simulink library "sm_wheel_loader_lib"  (R2025a)
settings: Solver=VariableStepAuto  StartTime=0.0  StopTime=10.0  RelTol=1e-3
undefined symbols (not defined in the file): AToTOrificeVector, BiPOrificeVector, boomHEArea, boomREArea, BToTOrificeVector, fluids, GRake, GToothL, GToothR, HMPST, HydFcnParams, logLoad, Position, PToAOrificeVector, PToBOrificeVector, RakeL, RakeR, testInput, Wheel_Loader, X, Y, Z
libraries: sm_lib x694, fl_lib x183, nesl_utility x74, SimscapeFluids_lib x62, sdl_lib x25, cvt_components_lib x25, simulink_extras x5, $bdroot x4, wheel_loader_contact_lib x4, ee_lib x2, SignalEditorBlockLib x1, batteryecm_lib x1
(part 9 of 26)

== system sm_wheel_loader_lib/Wheel Loader Vehicle/Load/Log ==
  Load : Inport
  Base : Subsystem  mask{TranslationCartesianOffset=base_location, RotationAngle=base_orientation}
      mask prompts: TranslationCartesianOffset "Location Base [x y z] (m)"; RotationAngle "Orientation Base (deg)"
      mask TypeOptions TranslationCartesianOffset:
      | Transform
      | Location Base/TranslationCartesianOffset
      mask TypeOptions RotationAngle:
      | Transform
      | Orient Base/RotationAngle
      mask Display: image('sm_wheel_loader_logbase_IMAGE.png')
  Bin : Subsystem  mask{TranslationCartesianOffset=bin_location, RotationAngle=bin_orientation}
      mask prompts: TranslationCartesianOffset "Bin Offset [x y z] (m)"; RotationAngle "Bin Orientation about z (deg)"
      mask TypeOptions TranslationCartesianOffset:
      | Transform
      | Location Base/TranslationCartesianOffset
      mask TypeOptions RotationAngle:
      | Transform
      | Orient Base/RotationAngle
      mask Display: image('sm_wheel_loader_logbin_IMAGE.png')
  Bushing Joint : sm_lib/Joints/Bushing Joint  JointMode=Normal  CompositeWrenchDir=FollowerOnBase  CompositeWrenchFrame=BaseFrame  SenseConstraintForce=off  SenseConstraintTorque=off  SenseTotalForce=off  SenseTotalTorque=off  PxPositionTargetSpecify=off  PxPositionTargetPriority=High  PxPositionTargetValue=0  PxPositionTargetValueUnits=m  PxVelocityTargetSpecify=off  PxVelocityTargetPriority=High  PxVelocityTargetValue=0  PxVelocityTargetValueUnits=m/s  PxEquilibriumPosition=0  PxEquilibriumPositionUnits=m  PxSpringStiffness=0  PxSpringStiffnessUnits=N/m  PxDampingCoefficient=0  PxDampingCoefficientUnits=N/(m/s)  PxLowerLimitSpecify=off  PxLowerLimitBound=-1  PxLowerLimitBoundUnits=m  PxLowerLimitStiffness=1e6  PxLowerLimitStiffnessUnits=N/m  PxLowerLimitDamping=1e3  PxLowerLimitDampingUnits=N/(m/s)  PxLowerLimitTransitionRegionWidth=1e-4  PxLowerLimitTransitionRegionWidthUnits=m  PxUpperLimitSpecify=off  PxUpperLimitBound=1  PxUpperLimitBoundUnits=m  PxUpperLimitStiffness=1e6  PxUpperLimitStiffnessUnits=N/m  PxUpperLimitDamping=1e3  PxUpperLimitDampingUnits=N/(m/s)  PxUpperLimitTransitionRegionWidth=1e-4  PxUpperLimitTransitionRegionWidthUnits=m  PxTorqueActuationMode=NoTorque  PxMotionActuationMode=ComputedMotion  PxSensePosition=off  PxSenseVelocity=off  PxSenseAcceleration=off  PxSenseTorqueForce=off  PxSenseLowerLimitTorqueForce=off  PxSenseUpperLimitTorqueForce=off  PyPositionTargetSpecify=off  PyPositionTargetPriority=High  PyPositionTargetValue=0  PyPositionTargetValueUnits=m  PyVelocityTargetSpecify=off  PyVelocityTargetPriority=High  PyVelocityTargetValue=0  PyVelocityTargetValueUnits=m/s  PyEquilibriumPosition=0  PyEquilibriumPositionUnits=m  PySpringStiffness=0  PySpringStiffnessUnits=N/m  PyDampingCoefficient=0  PyDampingCoefficientUnits=N/(m/s)  PyLowerLimitSpecify=off  PyLowerLimitBound=-1  PyLowerLimitBoundUnits=m  PyLowerLimitStiffness=1e6  PyLowerLimitStiffnessUnits=N/m  PyLowerLimitDamping=1e3  PyLowerLimitDampingUnits=N/(m/s)  PyLowerLimitTransitionRegionWidth=1e-4  PyLowerLimitTransitionRegionWidthUnits=m  PyUpperLimitSpecify=off  PyUpperLimitBound=1  PyUpperLimitBoundUnits=m  PyUpperLimitStiffness=1e6  PyUpperLimitStiffnessUnits=N/m  PyUpperLimitDamping=1e3  PyUpperLimitDampingUnits=N/(m/s)  PyUpperLimitTransitionRegionWidth=1e-4  PyUpperLimitTransitionRegionWidthUnits=m  PyTorqueActuationMode=NoTorque  PyMotionActuationMode=ComputedMotion  PySensePosition=off  PySenseVelocity=off  PySenseAcceleration=off  PySenseTorqueForce=off  PySenseLowerLimitTorqueForce=off  PySenseUpperLimitTorqueForce=off  PzPositionTargetSpecify=off  PzPositionTargetPriority=High  PzPositionTargetValue=0  PzPositionTargetValueUnits=m  PzVelocityTargetSpecify=off  PzVelocityTargetPriority=High  PzVelocityTargetValue=0  PzVelocityTargetValueUnits=m/s  PzEquilibriumPosition=0  PzEquilibriumPositionUnits=m  PzSpringStiffness=0  PzSpringStiffnessUnits=N/m  PzDampingCoefficient=0  PzDampingCoefficientUnits=N/(m/s)  PzLowerLimitSpecify=off  PzLowerLimitBound=-1  PzLowerLimitBoundUnits=m  PzLowerLimitStiffness=1e6  PzLowerLimitStiffnessUnits=N/m  PzLowerLimitDamping=1e3  PzLowerLimitDampingUnits=N/(m/s)  PzLowerLimitTransitionRegionWidth=1e-4  PzLowerLimitTransitionRegionWidthUnits=m  PzUpperLimitSpecify=off  PzUpperLimitBound=1  PzUpperLimitBoundUnits=m  PzUpperLimitStiffness=1e6  PzUpperLimitStiffnessUnits=N/m  PzUpperLimitDamping=1e3  PzUpperLimitDampingUnits=N/(m/s)  PzUpperLimitTransitionRegionWidth=1e-4  PzUpperLimitTransitionRegionWidthUnits=m  PzTorqueActuationMode=NoTorque  PzMotionActuationMode=ComputedMotion  PzSensePosition=off  PzSenseVelocity=off  PzSenseAcceleration=off  PzSenseTorqueForce=off  PzSenseLowerLimitTorqueForce=off  PzSenseUpperLimitTorqueForce=off  RxPositionTargetSpecify=off  RxPositionTargetPriority=High  RxPositionTargetValue=0  RxPositionTargetValueUnits=deg  RxVelocityTargetSpecify=off  RxVelocityTargetPriority=High  RxVelocityTargetValue=0  RxVelocityTargetValueUnits=deg/s  RxEquilibriumPosition=0  RxEquilibriumPositionUnits=deg  RxSpringStiffness=0  RxSpringStiffnessUnits=N*m/deg  RxDampingCoefficient=0  RxDampingCoefficientUnits=N*m/(deg/s)  RxLowerLimitSpecify=off  RxLowerLimitBound=-90  RxLowerLimitBoundUnits=deg  RxLowerLimitStiffness=1e4  RxLowerLimitStiffnessUnits=N*m/deg  RxLowerLimitDamping=10  RxLowerLimitDampingUnits=N*m/(deg/s)  RxLowerLimitTransitionRegionWidth=0.1  RxLowerLimitTransitionRegionWidthUnits=deg  RxUpperLimitSpecify=off  RxUpperLimitBound=90  RxUpperLimitBoundUnits=deg  RxUpperLimitStiffness=1e4  RxUpperLimitStiffnessUnits=N*m/deg  RxUpperLimitDamping=10  RxUpperLimitDampingUnits=N*m/(deg/s)  RxUpperLimitTransitionRegionWidth=0.1  RxUpperLimitTransitionRegionWidthUnits=deg  RxTorqueActuationMode=NoTorque  RxMotionActuationMode=ComputedMotion  RxSensePosition=off  RxSenseVelocity=off  RxSenseAcceleration=off  RxSenseTorqueForce=off  RxSenseLowerLimitTorqueForce=off  RxSenseUpperLimitTorqueForce=off  RyPositionTargetSpecify=off  RyPositionTargetPriority=High  RyPositionTargetValue=0  RyPositionTargetValueUnits=deg  RyVelocityTargetSpecify=off  RyVelocityTargetPriority=High  RyVelocityTargetValue=0  RyVelocityTargetValueUnits=deg/s  RyEquilibriumPosition=0  RyEquilibriumPositionUnits=deg  RySpringStiffness=0  RySpringStiffnessUnits=N*m/deg  RyDampingCoefficient=0  RyDampingCoefficientUnits=N*m/(deg/s)  RyLowerLimitSpecify=off  RyLowerLimitBound=-90  RyLowerLimitBoundUnits=deg  RyLowerLimitStiffness=1e4  RyLowerLimitStiffnessUnits=N*m/deg  RyLowerLimitDamping=10  RyLowerLimitDampingUnits=N*m/(deg/s)  RyLowerLimitTransitionRegionWidth=0.1  RyLowerLimitTransitionRegionWidthUnits=deg  RyUpperLimitSpecify=off  RyUpperLimitBound=90  RyUpperLimitBoundUnits=deg  RyUpperLimitStiffness=1e4  RyUpperLimitStiffnessUnits=N*m/deg  RyUpperLimitDamping=10  RyUpperLimitDampingUnits=N*m/(deg/s)  RyUpperLimitTransitionRegionWidth=0.1  RyUpperLimitTransitionRegionWidthUnits=deg  RyTorqueActuationMode=NoTorque  RyMotionActuationMode=ComputedMotion  RySensePosition=off  RySenseVelocity=off  RySenseAcceleration=off  RySenseTorqueForce=off  RySenseLowerLimitTorqueForce=off  RySenseUpperLimitTorqueForce=off  RzPositionTargetSpecify=off  RzPositionTargetPriority=High  RzPositionTargetValue=0  RzPositionTargetValueUnits=deg  RzVelocityTargetSpecify=off  RzVelocityTargetPriority=High  RzVelocityTargetValue=0  RzVelocityTargetValueUnits=deg/s  RzEquilibriumPosition=0  RzEquilibriumPositionUnits=deg  RzSpringStiffness=0  RzSpringStiffnessUnits=N*m/deg  RzDampingCoefficient=0  RzDampingCoefficientUnits=N*m/(deg/s)  RzLowerLimitSpecify=off  RzLowerLimitBound=-90  RzLowerLimitBoundUnits=deg  RzLowerLimitStiffness=1e4  RzLowerLimitStiffnessUnits=N*m/deg  RzLowerLimitDamping=10  RzLowerLimitDampingUnits=N*m/(deg/s)  RzLowerLimitTransitionRegionWidth=0.1  RzLowerLimitTransitionRegionWidthUnits=deg  RzUpperLimitSpecify=off  RzUpperLimitBound=90  RzUpperLimitBoundUnits=deg  RzUpperLimitStiffness=1e4  RzUpperLimitStiffnessUnits=N*m/deg  RzUpperLimitDamping=10  RzUpperLimitDampingUnits=N*m/(deg/s)  RzUpperLimitTransitionRegionWidth=0.1  RzUpperLimitTransitionRegionWidthUnits=deg  RzTorqueActuationMode=NoTorque  RzMotionActuationMode=ComputedMotion  RzSensePosition=off  RzSenseVelocity=off  RzSenseAcceleration=off  RzSenseTorqueForce=off  RzSenseLowerLimitTorqueForce=off  RzSenseUpperLimitTorqueForce=off
  Contact Force Base L : sm_lib/Forces and Torques/Spatial Contact Force  SenseSeparationDistance=off  NormalForceType=SmoothSpringDamper  NormalStiffness=logLoad.Contact.Base.stiffness  NormalStiffnessUnits=N/m  NormalDamping=logLoad.Contact.Base.damping  NormalDampingUnits=N/(m/s)  NormalTransitionRegionWidth=logLoad.Contact.Base.transRegWidth  NormalTransitionRegionWidthUnits=m  FrictionType=SmoothStickSlip  CoefficientOfStaticFriction=logLoad.Contact.Base.muStatic  CoefficientOfDynamicFriction=logLoad.Contact.Base.muDynamic  FrictionalCriticalVelocity=logLoad.Contact.Base.velThreshold  FrictionalCriticalVelocityUnits=m/s  SenseContactSignal=off  SensePenetrationDepth=off  SenseNormalVelocity=off  SenseTangentialVelocity=off  SensingForceTorqueDirection=BaseOnFollower  SensingForceTorqueResolutionFrame=ContactFrame  SenseNormalForce=off  SenseNormalForceMagnitude=off  SenseNormalTorque=off  SenseFrictionalForce=off  SenseFrictionalForceMagnitude=off  SenseFrictionalTorque=off  SenseTotalForce=off  SenseTotalTorque=off  SenseContactBaseRotation=off  SenseContactBaseTranslation=off  SenseContactFollowerRotation=off  SenseContactFollowerTranslation=off  ZeroCrossDetectContactStartAndEnd=off
  Contact Force Base R : sm_lib/Forces and Torques/Spatial Contact Force  SenseSeparationDistance=off  NormalForceType=SmoothSpringDamper  NormalStiffness=logLoad.Contact.Base.stiffness  NormalStiffnessUnits=N/m  NormalDamping=logLoad.Contact.Base.damping  NormalDampingUnits=N/(m/s)  NormalTransitionRegionWidth=logLoad.Contact.Base.transRegWidth  NormalTransitionRegionWidthUnits=m  FrictionType=SmoothStickSlip  CoefficientOfStaticFriction=logLoad.Contact.Base.muStatic  CoefficientOfDynamicFriction=logLoad.Contact.Base.muDynamic  FrictionalCriticalVelocity=logLoad.Contact.Base.velThreshold  FrictionalCriticalVelocityUnits=m/s  SenseContactSignal=off  SensePenetrationDepth=off  SenseNormalVelocity=off  SenseTangentialVelocity=off  SensingForceTorqueDirection=BaseOnFollower  SensingForceTorqueResolutionFrame=ContactFrame  SenseNormalForce=off  SenseNormalForceMagnitude=off  SenseNormalTorque=off  SenseFrictionalForce=off  SenseFrictionalForceMagnitude=off  SenseFrictionalTorque=off  SenseTotalForce=off  SenseTotalTorque=off  SenseContactBaseRotation=off  SenseContactBaseTranslation=off  SenseContactFollowerRotation=off  SenseContactFollowerTranslation=off  ZeroCrossDetectContactStartAndEnd=off
  Contact Force LogL BinA : sm_lib/Forces and Torques/Spatial Contact Force  SenseSeparationDistance=off  NormalForceType=SmoothSpringDamper  NormalStiffness=logLoad.Contact.Bin.stiffness  NormalStiffnessUnits=N/m  NormalDamping=logLoad.Contact.Bin.damping  NormalDampingUnits=N/(m/s)  NormalTransitionRegionWidth=logLoad.Contact.Bin.transRegWidth  NormalTransitionRegionWidthUnits=m  FrictionType=SmoothStickSlip  CoefficientOfStaticFriction=logLoad.Contact.Bin.muStatic  CoefficientOfDynamicFriction=logLoad.Contact.Bin.muDynamic  FrictionalCriticalVelocity=logLoad.Contact.Bin.velThreshold  FrictionalCriticalVelocityUnits=m/s  SenseContactSignal=off  SensePenetrationDepth=off  SenseNormalVelocity=off  SenseTangentialVelocity=off  SensingForceTorqueDirection=BaseOnFollower  SensingForceTorqueResolutionFrame=ContactFrame  SenseNormalForce=off  SenseNormalForceMagnitude=off  SenseNormalTorque=off  SenseFrictionalForce=off  SenseFrictionalForceMagnitude=off  SenseFrictionalTorque=off  SenseTotalForce=off  SenseTotalTorque=off  SenseContactBaseRotation=off  SenseContactBaseTranslation=off  SenseContactFollowerRotation=off  SenseContactFollowerTranslation=off  ZeroCrossDetectContactStartAndEnd=off
  Contact Force LogL BinA1 : sm_lib/Forces and Torques/Spatial Contact Force  SenseSeparationDistance=off  NormalForceType=SmoothSpringDamper  NormalStiffness=logLoad.Contact.Bin.stiffness  NormalStiffnessUnits=N/m  NormalDamping=logLoad.Contact.Bin.damping  NormalDampingUnits=N/(m/s)  NormalTransitionRegionWidth=logLoad.Contact.Bin.transRegWidth  NormalTransitionRegionWidthUnits=m  FrictionType=SmoothStickSlip  CoefficientOfStaticFriction=logLoad.Contact.Bin.muStatic  CoefficientOfDynamicFriction=logLoad.Contact.Bin.muDynamic  FrictionalCriticalVelocity=logLoad.Contact.Bin.velThreshold  FrictionalCriticalVelocityUnits=m/s  SenseContactSignal=off  SensePenetrationDepth=off  SenseNormalVelocity=off  SenseTangentialVelocity=off  SensingForceTorqueDirection=BaseOnFollower  SensingForceTorqueResolutionFrame=ContactFrame  SenseNormalForce=off  SenseNormalForceMagnitude=off  SenseNormalTorque=off  SenseFrictionalForce=off  SenseFrictionalForceMagnitude=off  SenseFrictionalTorque=off  SenseTotalForce=off  SenseTotalTorque=off  SenseContactBaseRotation=off  SenseContactBaseTranslation=off  SenseContactFollowerRotation=off  SenseContactFollowerTranslation=off  ZeroCrossDetectContactStartAndEnd=off
  Contact Force LogL Gnd : sm_lib/Forces and Torques/Spatial Contact Force  SenseSeparationDistance=off  NormalForceType=SmoothSpringDamper  NormalStiffness=logLoad.Contact.Surface.stiffness  NormalStiffnessUnits=N/m  NormalDamping=logLoad.Contact.Surface.damping  NormalDampingUnits=N/(m/s)  NormalTransitionRegionWidth=logLoad.Contact.Surface.transRegWidth  NormalTransitionRegionWidthUnits=m  FrictionType=SmoothStickSlip  CoefficientOfStaticFriction=logLoad.Contact.Surface.muStatic  CoefficientOfDynamicFriction=logLoad.Contact.Surface.muDynamic  FrictionalCriticalVelocity=logLoad.Contact.Surface.velThreshold  FrictionalCriticalVelocityUnits=m/s  SenseContactSignal=off  SensePenetrationDepth=off  SenseNormalVelocity=off  SenseTangentialVelocity=off  SensingForceTorqueDirection=BaseOnFollower  SensingForceTorqueResolutionFrame=ContactFrame  SenseNormalForce=off  SenseNormalForceMagnitude=off  SenseNormalTorque=off  SenseFrictionalForce=off  SenseFrictionalForceMagnitude=off  SenseFrictionalTorque=off  SenseTotalForce=off  SenseTotalTorque=off  SenseContactBaseRotation=off  SenseContactBaseTranslation=off  SenseContactFollowerRotation=off  SenseContactFollowerTranslation=off  ZeroCrossDetectContactStartAndEnd=off
  Contact Force LogR Gnd : sm_lib/Forces and Torques/Spatial Contact Force  SenseSeparationDistance=off  NormalForceType=SmoothSpringDamper  NormalStiffness=logLoad.Contact.Surface.stiffness  NormalStiffnessUnits=N/m  NormalDamping=logLoad.Contact.Surface.damping  NormalDampingUnits=N/(m/s)  NormalTransitionRegionWidth=logLoad.Contact.Surface.transRegWidth  NormalTransitionRegionWidthUnits=m  FrictionType=SmoothStickSlip  CoefficientOfStaticFriction=logLoad.Contact.Surface.muStatic  CoefficientOfDynamicFriction=logLoad.Contact.Surface.muDynamic  FrictionalCriticalVelocity=logLoad.Contact.Surface.velThreshold  FrictionalCriticalVelocityUnits=m/s  SenseContactSignal=off  SensePenetrationDepth=off  SenseNormalVelocity=off  SenseTangentialVelocity=off  SensingForceTorqueDirection=BaseOnFollower  SensingForceTorqueResolutionFrame=ContactFrame  SenseNormalForce=off  SenseNormalForceMagnitude=off  SenseNormalTorque=off  SenseFrictionalForce=off  SenseFrictionalForceMagnitude=off  SenseFrictionalTorque=off  SenseTotalForce=off  SenseTotalTorque=off  SenseContactBaseRotation=off  SenseContactBaseTranslation=off  SenseContactFollowerRotation=off  SenseContactFollowerTranslation=off  ZeroCrossDetectContactStartAndEnd=off
  Contact Force LogR GndA : sm_lib/Forces and Torques/Spatial Contact Force  SenseSeparationDistance=off  NormalForceType=SmoothSpringDamper  NormalStiffness=logLoad.Contact.Bin.stiffness  NormalStiffnessUnits=N/m  NormalDamping=logLoad.Contact.Bin.damping  NormalDampingUnits=N/(m/s)  NormalTransitionRegionWidth=logLoad.Contact.Bin.transRegWidth  NormalTransitionRegionWidthUnits=m  FrictionType=SmoothStickSlip  CoefficientOfStaticFriction=logLoad.Contact.Bin.muStatic  CoefficientOfDynamicFriction=logLoad.Contact.Bin.muDynamic  FrictionalCriticalVelocity=logLoad.Contact.Bin.velThreshold  FrictionalCriticalVelocityUnits=m/s  SenseContactSignal=off  SensePenetrationDepth=off  SenseNormalVelocity=off  SenseTangentialVelocity=off  SensingForceTorqueDirection=BaseOnFollower  SensingForceTorqueResolutionFrame=ContactFrame  SenseNormalForce=off  SenseNormalForceMagnitude=off  SenseNormalTorque=off  SenseFrictionalForce=off  SenseFrictionalForceMagnitude=off  SenseFrictionalTorque=off  SenseTotalForce=off  SenseTotalTorque=off  SenseContactBaseRotation=off  SenseContactBaseTranslation=off  SenseContactFollowerRotation=off  SenseContactFollowerTranslation=off  ZeroCrossDetectContactStartAndEnd=off
  Contact Force LogR GndB : sm_lib/Forces and Torques/Spatial Contact Force  SenseSeparationDistance=off  NormalForceType=SmoothSpringDamper  NormalStiffness=logLoad.Contact.Bin.stiffness  NormalStiffnessUnits=N/m  NormalDamping=logLoad.Contact.Bin.damping  NormalDampingUnits=N/(m/s)  NormalTransitionRegionWidth=logLoad.Contact.Bin.transRegWidth  NormalTransitionRegionWidthUnits=m  FrictionType=SmoothStickSlip  CoefficientOfStaticFriction=logLoad.Contact.Bin.muStatic  CoefficientOfDynamicFriction=logLoad.Contact.Bin.muDynamic  FrictionalCriticalVelocity=logLoad.Contact.Bin.velThreshold  FrictionalCriticalVelocityUnits=m/s  SenseContactSignal=off  SensePenetrationDepth=off  SenseNormalVelocity=off  SenseTangentialVelocity=off  SensingForceTorqueDirection=BaseOnFollower  SensingForceTorqueResolutionFrame=ContactFrame  SenseNormalForce=off  SenseNormalForceMagnitude=off  SenseNormalTorque=off  SenseFrictionalForce=off  SenseFrictionalForceMagnitude=off  SenseFrictionalTorque=off  SenseTotalForce=off  SenseTotalTorque=off  SenseContactBaseRotation=off  SenseContactBaseTranslation=off  SenseContactFollowerRotation=off  SenseContactFollowerTranslation=off  ZeroCrossDetectContactStartAndEnd=off
  Contact Force Log Rake : sm_lib/Forces and Torques/Spatial Contact Force  SenseSeparationDistance=off  NormalForceType=SmoothSpringDamper  NormalStiffness=logLoad.Contact.Grapple.stiffness  NormalStiffnessUnits=N/m  NormalDamping=logLoad.Contact.Grapple.damping  NormalDampingUnits=N/(m/s)  NormalTransitionRegionWidth=logLoad.Contact.Grapple.transRegWidth  NormalTransitionRegionWidthUnits=m  FrictionType=SmoothStickSlip  CoefficientOfStaticFriction=logLoad.Contact.Grapple.muStatic  CoefficientOfDynamicFriction=logLoad.Contact.Grapple.muDynamic  FrictionalCriticalVelocity=logLoad.Contact.Grapple.velThreshold  FrictionalCriticalVelocityUnits=m/s  SenseContactSignal=off  SensePenetrationDepth=off  SenseNormalVelocity=off  SenseTangentialVelocity=off  SensingForceTorqueDirection=BaseOnFollower  SensingForceTorqueResolutionFrame=ContactFrame  SenseNormalForce=off  SenseNormalForceMagnitude=off  SenseNormalTorque=off  SenseFrictionalForce=off  SenseFrictionalForceMagnitude=off  SenseFrictionalTorque=off  SenseTotalForce=off  SenseTotalTorque=off  SenseContactBaseRotation=off  SenseContactBaseTranslation=off  SenseContactFollowerRotation=off  SenseContactFollowerTranslation=off  ZeroCrossDetectContactStartAndEnd=off
  Contact Force Log ToothL : sm_lib/Forces and Torques/Spatial Contact Force  SenseSeparationDistance=off  NormalForceType=SmoothSpringDamper  NormalStiffness=logLoad.Contact.Grapple.stiffness  NormalStiffnessUnits=N/m  NormalDamping=logLoad.Contact.Grapple.damping  NormalDampingUnits=N/(m/s)  NormalTransitionRegionWidth=logLoad.Contact.Grapple.transRegWidth  NormalTransitionRegionWidthUnits=m  FrictionType=SmoothStickSlip  CoefficientOfStaticFriction=logLoad.Contact.Grapple.muStatic  CoefficientOfDynamicFriction=logLoad.Contact.Grapple.muDynamic  FrictionalCriticalVelocity=logLoad.Contact.Grapple.velThreshold  FrictionalCriticalVelocityUnits=m/s  SenseContactSignal=off  SensePenetrationDepth=off  SenseNormalVelocity=off  SenseTangentialVelocity=off  SensingForceTorqueDirection=BaseOnFollower  SensingForceTorqueResolutionFrame=ContactFrame  SenseNormalForce=off  SenseNormalForceMagnitude=off  SenseNormalTorque=off  SenseFrictionalForce=off  SenseFrictionalForceMagnitude=off  SenseFrictionalTorque=off  SenseTotalForce=off  SenseTotalTorque=off  SenseContactBaseRotation=off  SenseContactBaseTranslation=off  SenseContactFollowerRotation=off  SenseContactFollowerTranslation=off  ZeroCrossDetectContactStartAndEnd=off
  Contact Force Log ToothR : sm_lib/Forces and Torques/Spatial Contact Force  SenseSeparationDistance=off  NormalForceType=SmoothSpringDamper  NormalStiffness=logLoad.Contact.Grapple.stiffness  NormalStiffnessUnits=N/m  NormalDamping=logLoad.Contact.Grapple.damping  NormalDampingUnits=N/(m/s)  NormalTransitionRegionWidth=logLoad.Contact.Grapple.transRegWidth  NormalTransitionRegionWidthUnits=m  FrictionType=SmoothStickSlip  CoefficientOfStaticFriction=logLoad.Contact.Grapple.muStatic  CoefficientOfDynamicFriction=logLoad.Contact.Grapple.muDynamic  FrictionalCriticalVelocity=logLoad.Contact.Grapple.velThreshold  FrictionalCriticalVelocityUnits=m/s  SenseContactSignal=off  SensePenetrationDepth=off  SenseNormalVelocity=off  SenseTangentialVelocity=off  SensingForceTorqueDirection=BaseOnFollower  SensingForceTorqueResolutionFrame=ContactFrame  SenseNormalForce=off  SenseNormalForceMagnitude=off  SenseNormalTorque=off  SenseFrictionalForce=off  SenseFrictionalForceMagnitude=off  SenseFrictionalTorque=off  SenseTotalForce=off  SenseTotalTorque=off  SenseContactBaseRotation=off  SenseContactBaseTranslation=off  SenseContactFollowerRotation=off  SenseContactFollowerTranslation=off  ZeroCrossDetectContactStartAndEnd=off
  Log : Subsystem
      mask Display: image('sm_wheel_loader_log_IMAGE.png');
  Simscape Bus : SimscapeBus  HierarchyStrings=GToothL;GRake;GToothR
  Terminator : Terminator
  World Frame : sm_lib/Frames and Transforms/World Frame
  S : PMIOPort  Side=Left
  Im : PMIOPort  Port=2  Side=Left
  wires:
  Load/1 -> Terminator/1
  connections:
  Bushing Joint/RConn1 -- Log/RConn1
  Log/LConn3 -- Contact Force Base L/RConn1 -- Contact Force Log ToothR/RConn1 -- Contact Force Log Rake/RConn1 -- Contact Force Log ToothL/RConn1 -- Contact Force Base R/RConn1
  Contact Force LogR Gnd/RConn1 -- Log/LConn2 -- Contact Force LogR GndA/RConn1 -- Contact Force LogR GndB/RConn1
  Base/RConn3 -- Contact Force Base R/LConn1
  Bushing Joint/LConn1 -- Base/RConn2
  Contact Force Base L/LConn1 -- Base/RConn1
  Bin/RConn1 -- Contact Force LogR GndA/LConn1 -- Contact Force LogL BinA/LConn1
  Bin/RConn2 -- Contact Force LogL BinA1/LConn1 -- Contact Force LogR GndB/LConn1
  Contact Force LogL Gnd/RConn1 -- Log/LConn1 -- Contact Force LogL BinA1/RConn1 -- Contact Force LogL BinA/RConn1
  Im/RConn1 -- Simscape Bus/RConn1
  Contact Force LogL Gnd/LConn1 -- Contact Force LogR Gnd/LConn1 -- S/RConn1
  Contact Force Log ToothR/LConn1 -- Simscape Bus/LConn3
  Simscape Bus/LConn1 -- Contact Force Log ToothL/LConn1
  Contact Force Log Rake/LConn1 -- Simscape Bus/LConn2
  Base/LConn1 -- Bin/LConn1 -- World Frame/RConn1

== system sm_wheel_loader_lib/Wheel Loader Vehicle/Load/None ==
  Load : Inport
  Simscape Bus : SimscapeBus  HierarchyStrings=GToothL;GRake;GToothR
  Terminator : Terminator
  S : PMIOPort  Side=Left
  Im : PMIOPort  Port=2  Side=Left
  wires:
  Load/1 -> Terminator/1
  connections:
  Im/RConn1 -- Simscape Bus/RConn1

== system sm_wheel_loader_lib/Wheel Loader Vehicle/Steering Actuator/Actuator ==
  p : Inport
  Position : Subsystem  Tag=6d0be764-062f-4e0f-ba00-89e7ccc1dc31  VariantControl=Position
      mask Display: image('sm_wheel_loader_cyljoint_Position_IMAGE.png')
  Shaft : Subsystem  Tag=6d0be764-062f-4e0f-ba00-89e7ccc1dc31  VariantControl=Shaft
      mask Display: image('sm_wheel_loader_cyljoint_Shaft_IMAGE.png')
  R : PMIOPort  Side=Left
  B : PMIOPort  Port=2  Side=Left
  F : PMIOPort  Port=3  Side=Right
  m : Outport

== system sm_wheel_loader_lib/Wheel Loader Vehicle/Steering Actuator/Cylinder ==
  Collar : sm_lib/Body Elements/File Solid  ExtGeomFileName=Steer_Act_Cylinder_Collar.STEP  UnitType=FromFile  ExtGeomFileUnits=m  StepReaderType=HEX  ExportConvexHullGeometry=off  InertiaType=Custom  BasedOnType=DensityFromFile  Density=1000  DensityUnits=kg/m^3  Mass=Wheel_Loader.bodyGroups(50).subGroups(3).inertialProperties.mass  MassUnits=kg  CenterOfMass=Wheel_Loader.bodyGroups(50).subGroups(3).inertialProperties.centerOfMass  CenterOfMassUnits=m  MomentsOfInertia=Wheel_Loader.bodyGroups(50).subGroups(3).inertialProperties.momentsOfInertia  MomentsOfInertiaUnits=kg*m^2  ProductsOfInertia=Wheel_Loader.bodyGroups(50).subGroups(3).inertialProperties.productsOfInertia  ProductsOfInertiaUnits=kg*m^2  GraphicType=FromGeometry  MarkerShape=Sphere  MarkerSize=10  GraphicVisPropType=SimpleVisualProperties  GraphicDiffuseColor=Wheel_Loader.bodyGroups(50).subGroups(3).visualProperties.rgb  GraphicOpacity=Wheel_Loader.bodyGroups(50).subGroups(3).visualProperties.opacity  GraphicSpecularColor=[0.5 0.5 0.5 1.0]  GraphicAmbientColor=[0.15 0.15 0.15 1.0]  GraphicEmissiveColor=[0.0 0.0 0.0 1.0]  GraphicShininess=75  DoExposeReferenceFrame=on  SerializedFrames=<Frames/>
  Cylinder : sm_lib/Body Elements/File Solid  ExtGeomFileName=Steer_Act_Cylinder.STEP  UnitType=FromFile  ExtGeomFileUnits=m  StepReaderType=HEX  ExportConvexHullGeometry=off  InertiaType=Custom  BasedOnType=DensityFromFile  Density=1000  DensityUnits=kg/m^3  Mass=Wheel_Loader.bodyGroups(50).subGroups(1).inertialProperties.mass  MassUnits=kg  CenterOfMass=Wheel_Loader.bodyGroups(50).subGroups(1).inertialProperties.centerOfMass  CenterOfMassUnits=m  MomentsOfInertia=Wheel_Loader.bodyGroups(50).subGroups(1).inertialProperties.momentsOfInertia  MomentsOfInertiaUnits=kg*m^2  ProductsOfInertia=Wheel_Loader.bodyGroups(50).subGroups(1).inertialProperties.productsOfInertia  ProductsOfInertiaUnits=kg*m^2  GraphicType=FromGeometry  MarkerShape=Sphere  MarkerSize=10  GraphicVisPropType=SimpleVisualProperties  GraphicDiffuseColor=Wheel_Loader.bodyGroups(50).subGroups(1).visualProperties.rgb  GraphicOpacity=Wheel_Loader.bodyGroups(50).subGroups(1).visualProperties.opacity  GraphicSpecularColor=[0.5 0.5 0.5 1.0]  GraphicAmbientColor=[0.15 0.15 0.15 1.0]  GraphicEmissiveColor=[0.0 0.0 0.0 1.0]  GraphicShininess=75  DoExposeReferenceFrame=on  SerializedFrames=<Frames/>
  RT_RearFrame_SteeringActCyl : sm_lib/Frames and Transforms/Rigid Transform  RotationMethod=RotationMatrix  FollAlignAxisA=+X  BaseAlignAxisA=+Y  FollAlignAxisB=+Y  BaseAlignAxisB=+Z  RotationStandardAxis=+Z  RotationAngle=0.0  RotationAngleUnits=deg  RotationArbitraryAxis=[0 0 1]  RotationSequenceAxes=FollowerAxes  RotationSequence=XYX  RotationSequenceAngles=[0 0 0]  RotationSequenceAnglesUnits=deg  RotationMatrix=Wheel_Loader.coordSys(23).transform.rotation  Quaternion=[1 0 0 0]  TranslationMethod=Cartesian  TranslationCartesianOffset=Wheel_Loader.coordSys(23).transform.translation  TranslationCartesianOffsetUnits=m  TranslationStandardAxis=+Z  TranslationStandardOffset=0  TranslationStandardOffsetUnits=m  TranslationROffset=0  TranslationROffsetUnits=m  TranslationThetaOffset=0  TranslationThetaOffsetUnits=deg  TranslationZOffset=0  TranslationZOffsetUnits=m
  RT_Steering_Actuator : sm_lib/Frames and Transforms/Rigid Transform  RotationMethod=RotationMatrix  FollAlignAxisA=+X  BaseAlignAxisA=+Y  FollAlignAxisB=+Y  BaseAlignAxisB=+Z  RotationStandardAxis=+Z  RotationAngle=0.0  RotationAngleUnits=deg  RotationArbitraryAxis=[0 0 1]  RotationSequenceAxes=FollowerAxes  RotationSequence=XYX  RotationSequenceAngles=[0 0 0]  RotationSequenceAnglesUnits=deg  RotationMatrix=Wheel_Loader.coordSys(24).transform.rotation  Quaternion=[1 0 0 0]  TranslationMethod=Cartesian  TranslationCartesianOffset=Wheel_Loader.coordSys(24).transform.translation  TranslationCartesianOffsetUnits=m  TranslationStandardAxis=+Z  TranslationStandardOffset=0  TranslationStandardOffsetUnits=m  TranslationROffset=0  TranslationROffsetUnits=m  TranslationThetaOffset=0  TranslationThetaOffsetUnits=deg  TranslationZOffset=0  TranslationZOffsetUnits=m
  RT_Steering_Actuator_Offset : sm_lib/Frames and Transforms/Rigid Transform  RotationMethod=None  FollAlignAxisA=+X  BaseAlignAxisA=+Y  FollAlignAxisB=+Y  BaseAlignAxisB=+Z  RotationStandardAxis=+Z  RotationAngle=0.0  RotationAngleUnits=deg  RotationArbitraryAxis=[0 0 1]  RotationSequenceAxes=FollowerAxes  RotationSequence=XYX  RotationSequenceAngles=[0 0 0]  RotationSequenceAnglesUnits=deg  RotationMatrix=[1 0 0; 0 1 0; 0 0 1]  Quaternion=[1 0 0 0]  TranslationMethod=StandardAxis  TranslationCartesianOffset=[0 0 0]  TranslationCartesianOffsetUnits=m  TranslationStandardAxis=+Z  TranslationStandardOffset=HydFcnParams.steerActuator.mechModelCylOffset  TranslationStandardOffsetUnits=mm  TranslationROffset=0  TranslationROffsetUnits=m  TranslationThetaOffset=0  TranslationThetaOffsetUnits=deg  TranslationZOffset=0  TranslationZOffsetUnits=m
  Seal : sm_lib/Body Elements/File Solid  ExtGeomFileName=Steer_Act_Cylinder_Seal.STEP  UnitType=FromFile  ExtGeomFileUnits=m  StepReaderType=HEX  ExportConvexHullGeometry=off  InertiaType=Custom  BasedOnType=DensityFromFile  Density=1000  DensityUnits=kg/m^3  Mass=Wheel_Loader.bodyGroups(50).subGroups(2).inertialProperties.mass  MassUnits=kg  CenterOfMass=Wheel_Loader.bodyGroups(50).subGroups(2).inertialProperties.centerOfMass  CenterOfMassUnits=m  MomentsOfInertia=Wheel_Loader.bodyGroups(50).subGroups(2).inertialProperties.momentsOfInertia  MomentsOfInertiaUnits=kg*m^2  ProductsOfInertia=Wheel_Loader.bodyGroups(50).subGroups(2).inertialProperties.productsOfInertia  ProductsOfInertiaUnits=kg*m^2  GraphicType=FromGeometry  MarkerShape=Sphere  MarkerSize=10  GraphicVisPropType=SimpleVisualProperties  GraphicDiffuseColor=Wheel_Loader.bodyGroups(50).subGroups(2).visualProperties.rgb  GraphicOpacity=Wheel_Loader.bodyGroups(50).subGroups(2).visualProperties.opacity  GraphicSpecularColor=[0.5 0.5 0.5 1.0]  GraphicAmbientColor=[0.15 0.15 0.15 1.0]  GraphicEmissiveColor=[0.0 0.0 0.0 1.0]  GraphicShininess=75  DoExposeReferenceFrame=on  SerializedFrames=<Frames/>
  B : PMIOPort  Side=Left
  F : PMIOPort  Port=2  Side=Right
  connections:
  Seal/RConn1 -- Collar/RConn1 -- Cylinder/RConn1 -- RT_RearFrame_SteeringActCyl/LConn1 -- RT_Steering_Actuator/LConn1
  RT_RearFrame_SteeringActCyl/RConn1 -- B/RConn1
  RT_Steering_Actuator_Offset/RConn1 -- F/RConn1
  RT_Steering_Actuator/RConn1 -- RT_Steering_Actuator_Offset/LConn1

== system sm_wheel_loader_lib/Wheel Loader Vehicle/Steering Actuator/Rod ==
  Collar : sm_lib/Body Elements/File Solid  ExtGeomFileName=Steer_Act_Rod_Collar.STEP  UnitType=FromFile  ExtGeomFileUnits=m  StepReaderType=HEX  ExportConvexHullGeometry=off  InertiaType=Custom  BasedOnType=DensityFromFile  Density=1000  DensityUnits=kg/m^3  Mass=Wheel_Loader.bodyGroups(51).subGroups(2).inertialProperties.mass  MassUnits=kg  CenterOfMass=Wheel_Loader.bodyGroups(51).subGroups(2).inertialProperties.centerOfMass  CenterOfMassUnits=m  MomentsOfInertia=Wheel_Loader.bodyGroups(51).subGroups(2).inertialProperties.momentsOfInertia  MomentsOfInertiaUnits=kg*m^2  ProductsOfInertia=Wheel_Loader.bodyGroups(51).subGroups(2).inertialProperties.productsOfInertia  ProductsOfInertiaUnits=kg*m^2  GraphicType=FromGeometry  MarkerShape=Sphere  MarkerSize=10  GraphicVisPropType=SimpleVisualProperties  GraphicDiffuseColor=Wheel_Loader.bodyGroups(51).subGroups(2).visualProperties.rgb  GraphicOpacity=Wheel_Loader.bodyGroups(51).subGroups(2).visualProperties.opacity  GraphicSpecularColor=[0.5 0.5 0.5 1.0]  GraphicAmbientColor=[0.15 0.15 0.15 1.0]  GraphicEmissiveColor=[0.0 0.0 0.0 1.0]  GraphicShininess=75  DoExposeReferenceFrame=on  SerializedFrames=<Frames/>
  RT_SteeringActRod_FrontFrame : sm_lib/Frames and Transforms/Rigid Transform  RotationMethod=RotationMatrix  FollAlignAxisA=+X  BaseAlignAxisA=+Y  FollAlignAxisB=+Y  BaseAlignAxisB=+Z  RotationStandardAxis=+Z  RotationAngle=0.0  RotationAngleUnits=deg  RotationArbitraryAxis=[0 0 1]  RotationSequenceAxes=FollowerAxes  RotationSequence=XYX  RotationSequenceAngles=[0 0 0]  RotationSequenceAnglesUnits=deg  RotationMatrix=Wheel_Loader.coordSys(25).transform.rotation  Quaternion=[1 0 0 0]  TranslationMethod=Cartesian  TranslationCartesianOffset=Wheel_Loader.coordSys(25).transform.translation  TranslationCartesianOffsetUnits=m  TranslationStandardAxis=+Z  TranslationStandardOffset=0  TranslationStandardOffsetUnits=m  TranslationROffset=0  TranslationROffsetUnits=m  TranslationThetaOffset=0  TranslationThetaOffsetUnits=deg  TranslationZOffset=0  TranslationZOffsetUnits=m
  RT_Steering_Actuator : sm_lib/Frames and Transforms/Rigid Transform  RotationMethod=RotationMatrix  FollAlignAxisA=+X  BaseAlignAxisA=+Y  FollAlignAxisB=+Y  BaseAlignAxisB=+Z  RotationStandardAxis=+Z  RotationAngle=0.0  RotationAngleUnits=deg  RotationArbitraryAxis=[0 0 1]  RotationSequenceAxes=FollowerAxes  RotationSequence=XYX  RotationSequenceAngles=[0 0 0]  RotationSequenceAnglesUnits=deg  RotationMatrix=Wheel_Loader.coordSys(24).transform.rotation  Quaternion=[1 0 0 0]  TranslationMethod=Cartesian  TranslationCartesianOffset=Wheel_Loader.coordSys(24).transform.translation  TranslationCartesianOffsetUnits=m  TranslationStandardAxis=+Z  TranslationStandardOffset=0  TranslationStandardOffsetUnits=m  TranslationROffset=0  TranslationROffsetUnits=m  TranslationThetaOffset=0  TranslationThetaOffsetUnits=deg  TranslationZOffset=0  TranslationZOffsetUnits=m
  RT_Steering_Actuator_Offset : sm_lib/Frames and Transforms/Rigid Transform  RotationMethod=None  FollAlignAxisA=+X  BaseAlignAxisA=+Y  FollAlignAxisB=+Y  BaseAlignAxisB=+Z  RotationStandardAxis=+Z  RotationAngle=0.0  RotationAngleUnits=deg  RotationArbitraryAxis=[0 0 1]  RotationSequenceAxes=FollowerAxes  RotationSequence=XYX  RotationSequenceAngles=[0 0 0]  RotationSequenceAnglesUnits=deg  RotationMatrix=[1 0 0; 0 1 0; 0 0 1]  Quaternion=[1 0 0 0]  TranslationMethod=StandardAxis  TranslationCartesianOffset=[0 0 0]  TranslationCartesianOffsetUnits=m  TranslationStandardAxis=+Z  TranslationStandardOffset=HydFcnParams.steerActuator.mechModelRodOffset  TranslationStandardOffsetUnits=mm  TranslationROffset=0  TranslationROffsetUnits=m  TranslationThetaOffset=0  TranslationThetaOffsetUnits=deg  TranslationZOffset=0  TranslationZOffsetUnits=m
  Rod : sm_lib/Body Elements/File Solid  ExtGeomFileName=Steer_Act_Rod.STEP  UnitType=FromFile  ExtGeomFileUnits=m  StepReaderType=HEX  ExportConvexHullGeometry=off  InertiaType=Custom  BasedOnType=DensityFromFile  Density=1000  DensityUnits=kg/m^3  Mass=Wheel_Loader.bodyGroups(51).subGroups(1).inertialProperties.mass  MassUnits=kg  CenterOfMass=Wheel_Loader.bodyGroups(51).subGroups(1).inertialProperties.centerOfMass  CenterOfMassUnits=m  MomentsOfInertia=Wheel_Loader.bodyGroups(51).subGroups(1).inertialProperties.momentsOfInertia  MomentsOfInertiaUnits=kg*m^2  ProductsOfInertia=Wheel_Loader.bodyGroups(51).subGroups(1).inertialProperties.productsOfInertia  ProductsOfInertiaUnits=kg*m^2  GraphicType=FromGeometry  MarkerShape=Sphere  MarkerSize=10  GraphicVisPropType=SimpleVisualProperties  GraphicDiffuseColor=Wheel_Loader.bodyGroups(51).subGroups(1).visualProperties.rgb  GraphicOpacity=Wheel_Loader.bodyGroups(51).subGroups(1).visualProperties.opacity  GraphicSpecularColor=[0.5 0.5 0.5 1.0]  GraphicAmbientColor=[0.15 0.15 0.15 1.0]  GraphicEmissiveColor=[0.0 0.0 0.0 1.0]  GraphicShininess=75  DoExposeReferenceFrame=on  SerializedFrames=<Frames/>
  B : PMIOPort  Side=Left
  F : PMIOPort  Port=2  Side=Right
  connections:
  RT_Steering_Actuator/LConn1 -- Collar/RConn1 -- Rod/RConn1 -- RT_SteeringActRod_FrontFrame/LConn1
  RT_Steering_Actuator_Offset/RConn1 -- B/RConn1
  RT_SteeringActRod_FrontFrame/RConn1 -- F/RConn1
  RT_Steering_Actuator/RConn1 -- RT_Steering_Actuator_Offset/LConn1

== system sm_wheel_loader_lib/Controller/Desired Ratio Calc/HRB Control/PI HRB Brake ==
  error : Inport
  Rset : Inport  Port=2
  Gain : Gain  Gain=0.02*0.2
  Gain3 : Gain  Gain=0.002+0.0005
  Integrator : Integrator  ExternalReset=falling
  Sum : Sum  Inputs=++|
  ctrl : Outport
  wires:
  Rset/1 -> Integrator/2
  Integrator/1 -> Sum/1
  error/1 -> Gain3/1, Gain/1
  Sum/1 -> ctrl/1
  Gain3/1 -> Integrator/1
  Gain/1 -> Sum/2

== system sm_wheel_loader_lib/Controller/Desired Ratio Calc/HRB Control/PI HRB Regen ==
  error : Inport
  Rset : Inport  Port=2
  Gain : Gain  Gain=0.01*0.2
  Gain3 : Gain  Gain=0.001
  Integrator : Integrator  ExternalReset=falling
  Sum : Sum  Inputs=++|
  ctrl : Outport
  wires:
  Gain/1 -> Sum/2
  Gain3/1 -> Integrator/1
  Sum/1 -> ctrl/1
  error/1 -> Gain/1, Gain3/1
  Integrator/1 -> Sum/1
  Rset/1 -> Integrator/2

== system sm_wheel_loader_lib/Controller/Desired Ratio Calc/MB Control/PI MB No HRB ==
  error : Inport
  Rset : Inport  Port=2
  Gain : Gain  Gain=0.01
  Gain3 : Gain  Gain=0.002
  Integrator : Integrator  ExternalReset=falling
  Sum : Sum  Inputs=++|
  ctrl : Outport
  wires:
  Rset/1 -> Integrator/2
  Integrator/1 -> Sum/1
  error/1 -> Gain3/1, Gain/1
  Sum/1 -> ctrl/1
  Gain3/1 -> Integrator/1
  Gain/1 -> Sum/2

== system sm_wheel_loader_lib/Controller/Desired Ratio Calc/MB Control/PI MB with MRB ==
  error : Inport
  Rset : Inport  Port=2
  Gain : Gain  Gain=0.005
  Gain3 : Gain  Gain=0.002
  Integrator : Integrator  ExternalReset=falling
  Sum : Sum  Inputs=++|
  ctrl : Outport
  wires:
  Gain/1 -> Sum/2
  Gain3/1 -> Integrator/1
  Sum/1 -> ctrl/1
  error/1 -> Gain/1, Gain3/1
  Integrator/1 -> Sum/1
  Rset/1 -> Integrator/2

== system sm_wheel_loader_lib/Wheel Loader Vehicle/Actuators/Hydraulic/Actuator Linkage ==
  Actuator LiftL : SimscapeFluids_lib/Isothermal Liquid/Actuators/Double-Acting Actuator (IL)  single_fluid=true  mech_orientation=foundation.enum.MechOrientationTranslational.Positive  piston_area_A=HydFcnParams.liftActuator.headEndArea mm^2  piston_area_B=HydFcnParams.liftActuator.rodEndArea mm^2  stroke=HydFcnParams.liftActuator.stroke mm  dead_volume_A=1e-4 m^3  dead_volume_B=1e-4 m^3  pressure_spec=foundation.enum.pressure_spec.atmospheric  environment_pressure=0.101325 MPa  hardstop_model=simscape.enum.hardstop.smooth  stiff_coeff=1e8 N/m  damping_coeff=1e5 N/(m/s)  transition=0.1 mm  coeff_rest=0.7  v_tol=0.001 m/s  f_tol=0.001 N  cushion_A_spec=simscape.enum.onoff.off  area_plunger_A=boomHEArea/4 mm^2  length_plunger_A=5 mm  area_cushion_orifice_A=5 mm^2  area_leak_plunger_A=1e-7 m^2  p_crack_differential_A=0.01 MPa  press_max_differential_A=0.1 MPa  check_valve_area_max_A=1e-4 m^2  check_valve_area_leak_A=1e-10 m^2  smoothing_factor_A=0  cushion_B_spec=simscape.enum.onoff.off  area_plunger_B=boomREArea/4 mm^2  length_plunger_B=5 mm  area_cushion_orifice_B=5 mm^2  area_leak_plunger_B=1e-7 m^2  p_crack_differential_B=0.01 MPa  press_max_differential_B=0.1 MPa  check_valve_area_max_B=1e-4 m^2  check_valve_area_leak_B=1e-10 m^2  smoothing_factor_B=0  friction_spec=simscape.enum.onoff.on  breakaway_Coulomb_ratio=HydFcnParams.liftActuator.brkawyToCoulRatio  breakaway_velocity=HydFcnParams.liftActuator.brkawyVel m/s  preload_force=HydFcnParams.liftActuator.preloadForce N  Coulomb_coeff=HydFcnParams.liftActuator.coulForceCoef N/Pa  viscous_coeff=HydFcnParams.liftActuator.viscCoeff N/(m/s)  leakage_spec=simscape.enum.onoff.off  clearance=1e-4 m  piston_length=0.01 m  displacement_spec=foundation.enum.DisplacementSpec.Calculate  x0=testInput.Active.Lift.p(1)*1000 mm  dynamic_compressibility=simscape.enum.onoff.on  p0_A=HydFcnParams.liftActuator.initHEPr bar  p0_B=HydFcnParams.liftActuator.initREPr bar  p_nominal_A=0.101325 MPa  p_nominal_B=0.101325 MPa
      settings: InternalSimscapePortConfiguration="{\"Bottom\":[],\"Left\":[{\"id\":\"C\",\"label\":\"C\",\"type\":\"foundation.mechanical.translational.translational\"},{\"id\":\"A\",\"label\":\"A\",\"type\":\"foundation.isothermal_liquid.isothermal_liquid\"}],\"Right\":[{\"id\":\"p_out\",\"label\":\"p\",\"type\":\"output\"},{\"id\":\"R\",\"label\":\"R\",\"type\":\"foundation.mechanical.translational.translational\"},{\"id\":\"B\",\"label\":\"B\",\"type\":\"foundation.isothermal_liquid.isothermal_liquid\"}],\"Top\":[]}"
  Actuator LiftR : SimscapeFluids_lib/Isothermal Liquid/Actuators/Double-Acting Actuator (IL)  single_fluid=true  mech_orientation=foundation.enum.MechOrientationTranslational.Positive  piston_area_A=HydFcnParams.liftActuator.headEndArea mm^2  piston_area_B=HydFcnParams.liftActuator.rodEndArea mm^2  stroke=HydFcnParams.liftActuator.stroke mm  dead_volume_A=1e-4 m^3  dead_volume_B=1e-4 m^3  pressure_spec=foundation.enum.pressure_spec.atmospheric  environment_pressure=0.101325 MPa  hardstop_model=simscape.enum.hardstop.smooth  stiff_coeff=1e8 N/m  damping_coeff=1e5 N/(m/s)  transition=0.1 mm  coeff_rest=0.7  v_tol=0.001 m/s  f_tol=0.001 N  cushion_A_spec=simscape.enum.onoff.off  area_plunger_A=boomHEArea/4 mm^2  length_plunger_A=5 mm  area_cushion_orifice_A=5 mm^2  area_leak_plunger_A=1e-7 m^2  p_crack_differential_A=0.01 MPa  press_max_differential_A=0.1 MPa  check_valve_area_max_A=1e-4 m^2  check_valve_area_leak_A=1e-10 m^2  smoothing_factor_A=0  cushion_B_spec=simscape.enum.onoff.off  area_plunger_B=boomREArea/4 mm^2  length_plunger_B=5 mm  area_cushion_orifice_B=5 mm^2  area_leak_plunger_B=1e-7 m^2  p_crack_differential_B=0.01 MPa  press_max_differential_B=0.1 MPa  check_valve_area_max_B=1e-4 m^2  check_valve_area_leak_B=1e-10 m^2  smoothing_factor_B=0  friction_spec=simscape.enum.onoff.on  breakaway_Coulomb_ratio=HydFcnParams.liftActuator.brkawyToCoulRatio  breakaway_velocity=HydFcnParams.liftActuator.brkawyVel m/s  preload_force=HydFcnParams.liftActuator.preloadForce N  Coulomb_coeff=HydFcnParams.liftActuator.coulForceCoef N/Pa  viscous_coeff=HydFcnParams.liftActuator.viscCoeff N/(m/s)  leakage_spec=simscape.enum.onoff.off  clearance=1e-4 m  piston_length=0.01 m  displacement_spec=foundation.enum.DisplacementSpec.Calculate  x0=testInput.Active.Lift.p(1)*1000 mm  dynamic_compressibility=simscape.enum.onoff.on  p0_A=HydFcnParams.liftActuator.initHEPr bar  p0_B=HydFcnParams.liftActuator.initREPr bar  p_nominal_A=0.101325 MPa  p_nominal_B=0.101325 MPa
      settings: InternalSimscapePortConfiguration="{\"Bottom\":[],\"Left\":[{\"id\":\"C\",\"label\":\"C\",\"type\":\"foundation.mechanical.translational.translational\"},{\"id\":\"A\",\"label\":\"A\",\"type\":\"foundation.isothermal_liquid.isothermal_liquid\"}],\"Right\":[{\"id\":\"p_out\",\"label\":\"p\",\"type\":\"output\"},{\"id\":\"R\",\"label\":\"R\",\"type\":\"foundation.mechanical.translational.translational\"},{\"id\":\"B\",\"label\":\"B\",\"type\":\"foundation.isothermal_liquid.isothermal_liquid\"}],\"Top\":[]}"
  Actuator Tilt : SimscapeFluids_lib/Isothermal Liquid/Actuators/Double-Acting Actuator (IL)  single_fluid=true  mech_orientation=foundation.enum.MechOrientationTranslational.Positive  piston_area_A=HydFcnParams.tiltActuator.headEndArea mm^2  piston_area_B=HydFcnParams.tiltActuator.rodEndArea mm^2  stroke=HydFcnParams.tiltActuator.stroke mm  dead_volume_A=1e-4 m^3  dead_volume_B=1e-4 m^3  pressure_spec=foundation.enum.pressure_spec.atmospheric  environment_pressure=0.101325 MPa  hardstop_model=simscape.enum.hardstop.smooth  stiff_coeff=1e8 N/m  damping_coeff=1e5 N/(m/s)  transition=0.1 mm  coeff_rest=0.7  v_tol=0.001 m/s  f_tol=0.001 N  cushion_A_spec=simscape.enum.onoff.off  area_plunger_A=boomHEArea/4 mm^2  length_plunger_A=5 mm  area_cushion_orifice_A=5 mm^2  area_leak_plunger_A=1e-7 m^2  p_crack_differential_A=0.01 MPa  press_max_differential_A=0.1 MPa  check_valve_area_max_A=1e-4 m^2  check_valve_area_leak_A=1e-10 m^2  smoothing_factor_A=0  cushion_B_spec=simscape.enum.onoff.off  area_plunger_B=boomREArea/4 mm^2  length_plunger_B=5 mm  area_cushion_orifice_B=5 mm^2  area_leak_plunger_B=1e-7 m^2  p_crack_differential_B=0.01 MPa  press_max_differential_B=0.1 MPa  check_valve_area_max_B=1e-4 m^2  check_valve_area_leak_B=1e-10 m^2  smoothing_factor_B=0  friction_spec=true  breakaway_Coulomb_ratio=HydFcnParams.tiltActuator.brkawyToCoulRatio  breakaway_velocity=HydFcnParams.tiltActuator.brkawyVel m/s  preload_force=HydFcnParams.tiltActuator.preloadForce N  Coulomb_coeff=HydFcnParams.tiltActuator.coulForceCoef N/Pa  viscous_coeff=HydFcnParams.tiltActuator.viscCoeff lbf/(in/s)  leakage_spec=simscape.enum.onoff.off  clearance=1e-4 m  piston_length=0.01 m  displacement_spec=foundation.enum.DisplacementSpec.Calculate  x0=testInput.Active.Tilt.p(1)*1000 mm  dynamic_compressibility=simscape.enum.onoff.on  p0_A=HydFcnParams.tiltActuator.initHEPr bar  p0_B=HydFcnParams.tiltActuator.initREPr bar  p_nominal_A=0.101325 MPa  p_nominal_B=0.101325 MPa
      settings: InternalSimscapePortConfiguration="{\"Bottom\":[],\"Left\":[{\"id\":\"C\",\"label\":\"C\",\"type\":\"foundation.mechanical.translational.translational\"},{\"id\":\"A\",\"label\":\"A\",\"type\":\"foundation.isothermal_liquid.isothermal_liquid\"}],\"Right\":[{\"id\":\"p_out\",\"label\":\"p\",\"type\":\"output\"},{\"id\":\"R\",\"label\":\"R\",\"type\":\"foundation.mechanical.translational.translational\"},{\"id\":\"B\",\"label\":\"B\",\"type\":\"foundation.isothermal_liquid.isothermal_liquid\"}],\"Top\":[]}"
  MTRef Tilt : fl_lib/Mechanical/Translational Elements/Mechanical Translational Reference
  MTRef Tilt LiftR : fl_lib/Mechanical/Translational Elements/Mechanical Translational Reference
  MTRef TiltL : fl_lib/Mechanical/Translational Elements/Mechanical Translational Reference
  PS Terminator : fl_lib/Physical Signals/Sinks/PS Terminator
  PS Terminator1 : fl_lib/Physical Signals/Sinks/PS Terminator
  PS Terminator2 : fl_lib/Physical Signals/Sinks/PS Terminator
  LA : PMIOPort  Side=Left
  LB : PMIOPort  Port=2  Side=Left
  TA : PMIOPort  Port=3  Side=Left
  TB : PMIOPort  Port=4  Side=Left
  RLiftL : PMIOPort  Port=5  Side=Right
  RLiftR : PMIOPort  Port=6  Side=Right
  RTilt : PMIOPort  Port=7  Side=Right
  connections:
  Actuator Tilt/LConn2 -- TA/RConn1
  Actuator Tilt/RConn3 -- TB/RConn1
  RLiftR/RConn1 -- Actuator LiftR/RConn2
  Actuator LiftR/RConn3 -- Actuator LiftL/RConn3 -- LB/RConn1
  Actuator LiftR/LConn2 -- Actuator LiftL/LConn2 -- LA/RConn1
  Actuator LiftL/LConn1 -- MTRef TiltL/LConn1
  RLiftL/RConn1 -- Actuator LiftL/RConn2
  MTRef Tilt/LConn1 -- Actuator Tilt/LConn1
  RTilt/RConn1 -- Actuator Tilt/RConn2
  MTRef Tilt LiftR/LConn1 -- Actuator LiftR/LConn1
  Actuator LiftL/RConn1 -- PS Terminator/LConn1
  PS Terminator1/LConn1 -- Actuator LiftR/RConn1
  Actuator Tilt/RConn1 -- PS Terminator2/LConn1
